simulink model "five_cell_thermal_network"  (R2025b)
settings: Solver=ode45  StartTime=0.0  StopTime=2000  RelTol=1e-3
settings Model: Creator=Kayoky  LastModifiedBy=Kayoky

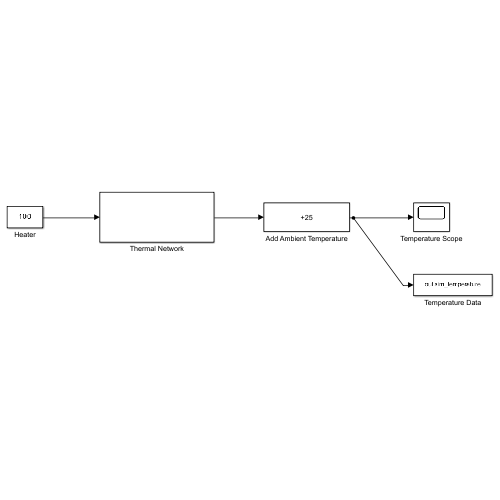
[thumbnail: Simulink's stored preview of the top-level diagram]
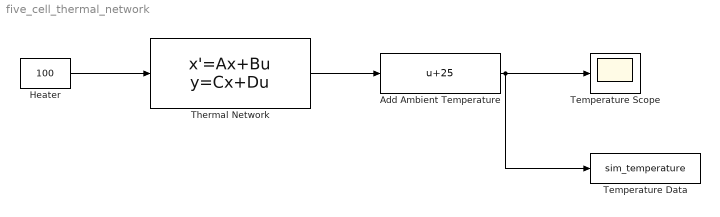
== system five_cell_thermal_network ==
  Add Ambient Temperature : Bias  Bias=25  SaturateOnIntegerOverflow=off
  Heater : Constant  Value=100
  Temperature Data : ToWorkspace  VariableName=sim_temperature  SaveFormat=Timeseries  SampleTime=-1
  Temperature Scope : Scope
  Thermal Network : StateSpace  A=[-0.000456554838709678 0.000161290322580645 0 0 0;0.000161290322580645 -0.000617845161290323 0.000161290322580645 0 0;0 0.000161290322580645 -0.000617845161290323 0.000161290322580645 0;0 0 0.000161290322580645 -0.000617845161290323 0.000161290322580645;0 0 0 0.000161290322580645 -0.000456554838709678]  B=[0.00032258064516129;0;0;0;0]  C=[1 0 0 0 0;0 1 0 0 0;0 0 1 0 0;0 0 0 1 0;0 0 0 0 1]  D=[0;0;0;0;0]  InitialCondition=zeros(5,1)
  wires:
  Heater/1 -> Thermal Network/1
  Thermal Network/1 -> Add Ambient Temperature/1
  Add Ambient Temperature/1 -> Temperature Scope/1, Temperature Data/1
